simulink model "experiment_supervisor_user"  (R2026b)
settings: Solver=FixedStepDiscrete  StopTime=inf
PreLoadFcn:
  | run('experiment_supervisor_data');
model workspace (MAT data in the model file):
  Ts = 0.0001
undefined symbols (not defined in the file or in its folder): ControlModes, MCControlModes, MCMotorParamsSet
libraries: dspswit3 x1, sldrtlib x1
settings Model: DataDictionary=amcmj1.sldd  SimulationMode=accelerator  Creator=mfussi  LastModifiedBy=ksangalli
settings OptimizationCC: DefaultUnderspecifiedDataType=single  GainParamInheritBuiltInType=on  ReuseModelBlockBuffer=off  SimCompilerOptimization=on
settings DebuggingCC: ParamSuppressDoubleToSinglePrecisionLossMsg=on
settings HardwareCC: ProdHWDeviceType=Intel->x86-64 (Linux 64)  ProdLongLongMode=on
settings RTWCC: DLArmComputeVersion=19.05  Description=Simulink Desktop Real-Time  RTWCompilerOptimization=on  SystemTargetFile=sldrt.tlc  TargetLang=C++  TemplateMakefile=sldrt.tmf
settings SimulinkDesktopRealTimeCC: OptimizeReductions=on  ParMdlRefBuildCompliant=on  RealTimeExecution=kernel  TargetLangStandard=C++11 (ISO)  TargetLibSuffix=_sldrt.a  TargetPreCompLibLocation=C:\Program Files\MATLAB\R2026b\toolbox\sldrt\lib\win64

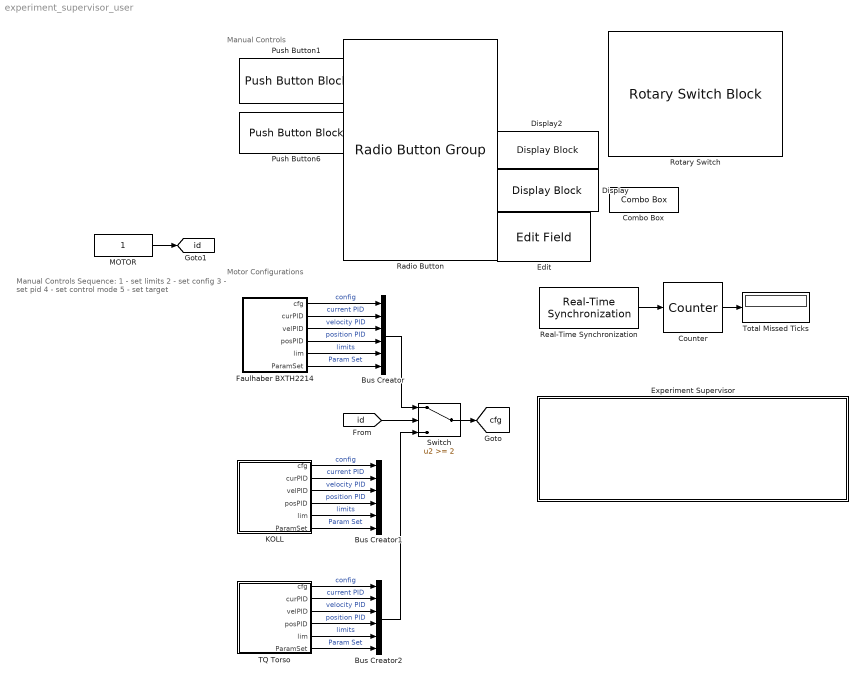
== system experiment_supervisor_user ==
  note: Manual Controls Sequence:
      | 1 - set limits
      | 2 - set config
      | 3 - set pid
      | 4 - set control mode
      | 5 - set target
  note: Motor Configurations
  note: Manual Controls
  Bus Creator : BusCreator  Inputs=6
  Bus Creator1 : BusCreator  Inputs=6
  Bus Creator2 : BusCreator  Inputs=6
  Combo Box : ComboBox  SelectedLabel=elect_vmax  UseEnumeratedDataType=on  EnumeratedDataType=MCMotorParamsSet
  Counter : dspswit3/Counter  Direction=Up  CountEvent=Rising edge  CounterSize=16 bits  MaxCount=10000  InitialCount=0  Output=Count  HitValue=32  ResetInput=off  SamplesPerFrame=1  Ts=1  CntDtype=uint16  HitDtype=Logical
  Display : DisplayBlock  Format=Integer  Transparency=1  GridColor=[1.0, 0.0, 0.0]
  Display2 : DisplayBlock  Format=Custom  Transparency=1  GridColor=[1.0, 0.0, 0.0]
  Edit : EditField  ShowInitialText=on  Alignment=Center
  Experiment Supervisor : Subsystem
  Faulhaber BXTH2214 : Subsystem
  KOLL : Subsystem
  MOTOR : Constant  OutDataTypeStr=uint32  SampleTime=0.01
  Push Button1 : PushButtonBlock  ButtonText=Send Polling CAN Msg  Icon=Triangle  IconAlignment=Right  IconOnColor=[1.0, 0.0, 1.0]  IconOffColor=[0.74901960784313726, 0.74901960784313726, 0.74901960784313726]  IconColor=On  OffValue=0.000000
  Push Button6 : PushButtonBlock  ButtonText=Send Streaming CAN Msg  ButtonType=Latch  Icon=TurnSignalRight  IconAlignment=Right  IconOnColor=[0.0, 0.0, 1.0]  IconOffColor=[0.74901960784313726, 0.74901960784313726, 0.74901960784313726]  IconColor=On  OffValue=0.000000
  Radio Button : RadioButtonGroup  LabelPosition=Hide  SelectedLabel=set-target  ButtonGroupName=Manual CAN Messages
  Real-Time Synchronization : sldrtlib/Real-Time Synchronization  SampleTime=Ts  MaxMissedTicks=inf  ShowMissedTicks=on  YieldWhenWaiting=off
  Rotary Switch : RotarySwitchBlock  LabelPosition=Hide  UseEnumeratedDataType=on  EnumeratedDataType=MCControlModes
  Switch : Switch  Threshold=2  SaturateOnIntegerOverflow=off  InputSameDT=off
  TQ Torso : Subsystem
  Total Missed Ticks : Display
      settings: Decimation=5
  tag scope: cfg=global, id=global
  wires:
  Real-Time Synchronization/1 -> Counter/1
  Faulhaber BXTH2214/1(cfg) -> Bus Creator/1  "config"
  Faulhaber BXTH2214/2(curPID) -> Bus Creator/2  "current PID"
  Faulhaber BXTH2214/3(velPID) -> Bus Creator/3  "velocity PID"
  Counter/1 -> Total Missed Ticks/1
  MOTOR/1 -> [id]
  Switch/1 -> [cfg]
  KOLL/1(cfg) -> Bus Creator1/1  "config"
  KOLL/2(curPID) -> Bus Creator1/2  "current PID"
  KOLL/3(velPID) -> Bus Creator1/3  "velocity PID"
  [id] -> Switch/2
  KOLL/5(lim) -> Bus Creator1/5  "limits"
  KOLL/4(posPID) -> Bus Creator1/4  "position PID"
  Faulhaber BXTH2214/4(posPID) -> Bus Creator/4  "position PID"
  Faulhaber BXTH2214/5(lim) -> Bus Creator/5  "limits"
  KOLL/6(ParamSet) -> Bus Creator1/6  "Param Set"
  Faulhaber BXTH2214/6(ParamSet) -> Bus Creator/6  "Param Set"
  Bus Creator/1 -> Switch/1
  TQ Torso/4(posPID) -> Bus Creator2/4  "position PID"
  TQ Torso/2(curPID) -> Bus Creator2/2  "current PID"
  TQ Torso/1(cfg) -> Bus Creator2/1  "config"
  TQ Torso/3(velPID) -> Bus Creator2/3  "velocity PID"
  TQ Torso/5(lim) -> Bus Creator2/5  "limits"
  TQ Torso/6(ParamSet) -> Bus Creator2/6  "Param Set"
  Bus Creator2/1 -> Switch/3

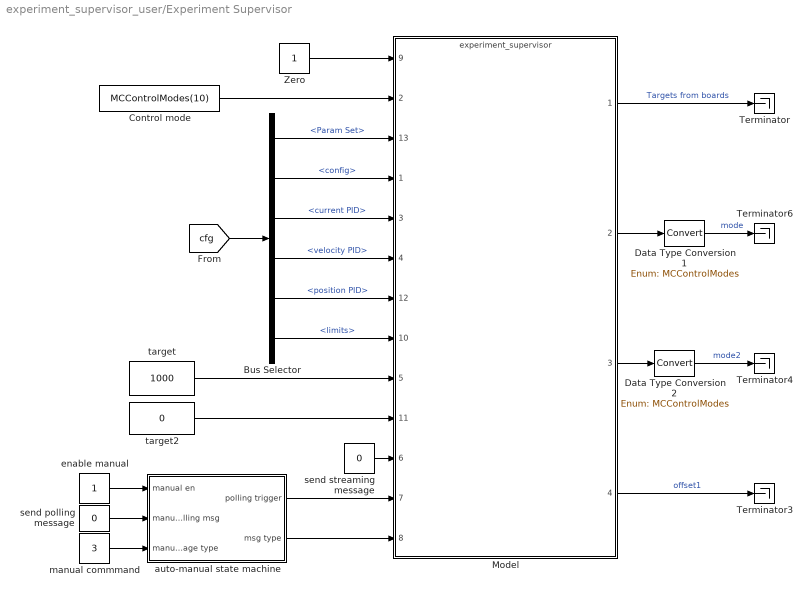
== system experiment_supervisor_user/Experiment Supervisor ==
  " Control mode" : Constant  Value=MCControlModes(10)
  Bus Selector : BusSelector  OutputSignals=Param Set,config,current PID,velocity PID,position PID,limits
  Data Type Conversion1 : DataTypeConversion  OutDataTypeStr=Enum: MCControlModes  SaturateOnIntegerOverflow=off  RndMeth=Floor
  Data Type Conversion2 : DataTypeConversion  OutDataTypeStr=Enum: MCControlModes  SaturateOnIntegerOverflow=off  RndMeth=Floor
  Model : ModelReference  ModelNameDialog=experiment_supervisor.slx  SimulationMode=Normal  ModelReferenceVersion=11.0
      settings: PortSchema="{\"entries\":[{\"content\":{\"sides\":[{\"content\":{\"connectorIds\":[\"In9\",\"In2\",\"In13\",\"In1\",\"In3\",\"In4\",\"In12\",\"In10\",\"In5\",\"In11\",\"In6\",\"In7\",\"In8\"]},\"type\":\"ConnectorPlacement.EquallySpacedRectSide\",\"uuid\":\"bfbdf898-42a5-495c-8a1e-d70d1f7414e8\"},{\"content\":{\"connectorIds\":[\"Out1\",\"Out2\",\"Out3\",\"Out4\"],\"side\":\"RIGHT\"},\"type\":\"ConnectorPlacement.EquallySpacedRectSide\",\"uuid\":\"3fb07422-e541-47fe-8bd2-34fc87b5d4e0\"},{\"content\":{\"side\":\"TOP\"},\"type\":\"ConnectorPlacement.EquallySpacedRectSide\",\"uuid\":\"cc070490-4dff-4736-882c-6ee4a91a824d\"}]},\"type\":\"ConnectorPlacement.EquallySpacedConnector\",\"uuid\":\"82f7e7bc-78f2-4fca-805f-7ff02feabc7a\"}],\"packageUris\":[\"http://schema.mathworks.com/mf0/Connector/R2020b\"],\"version\":\"1.0\"}"
  Terminator{,3..4,6} (4 alike) : Terminator
  Zero : Constant  OutDataTypeStr=Inherit: Inherit via back propagation
  auto-manual state machine : Subsystem
  enable manual : Constant  OutDataTypeStr=uint8
  manual commmand : Constant  Value=3  OutDataTypeStr=uint8
  send polling message : Constant  Value=0  OutDataTypeStr=uint8
  send streaming message : Constant  Value=0  OutDataTypeStr=Inherit: Inherit via back propagation
  target : Constant  Value=1000  OutDataTypeStr=single
  target2 : Constant  Value=0  OutDataTypeStr=single
  wires:
  Bus Selector/3 -> Model/3  "<current PID>"
  enable manual/1 -> auto-manual state machine/1(manual en)
  send polling message/1 -> auto-manual state machine/2(manual send polling msg)
  [cfg] -> Bus Selector/1
  manual commmand/1 -> auto-manual state machine/3(manual message type)
  " Control mode"/1 -> Model/2
  Bus Selector/2 -> Model/1  "<config>"
  Bus Selector/4 -> Model/4  "<velocity PID>"
  send streaming message/1 -> Model/6
  auto-manual state machine/1(polling trigger) -> Model/7
  Model/4 -> Terminator3/1  "offset1"
  auto-manual state machine/2(msg type) -> Model/8
  Model/1 -> Terminator/1  "Targets from boards"
  Model/2 -> Data Type Conversion1/1
  Data Type Conversion1/1 -> Terminator6/1  "mode"
  Zero/1 -> Model/9
  Data Type Conversion2/1 -> Terminator4/1  "mode2"
  Model/3 -> Data Type Conversion2/1
  target2/1 -> Model/11
  Bus Selector/5 -> Model/12  "<position PID>"
  target/1 -> Model/5
  Bus Selector/6 -> Model/10  "<limits>"
  Bus Selector/1 -> Model/13  "<Param Set>"

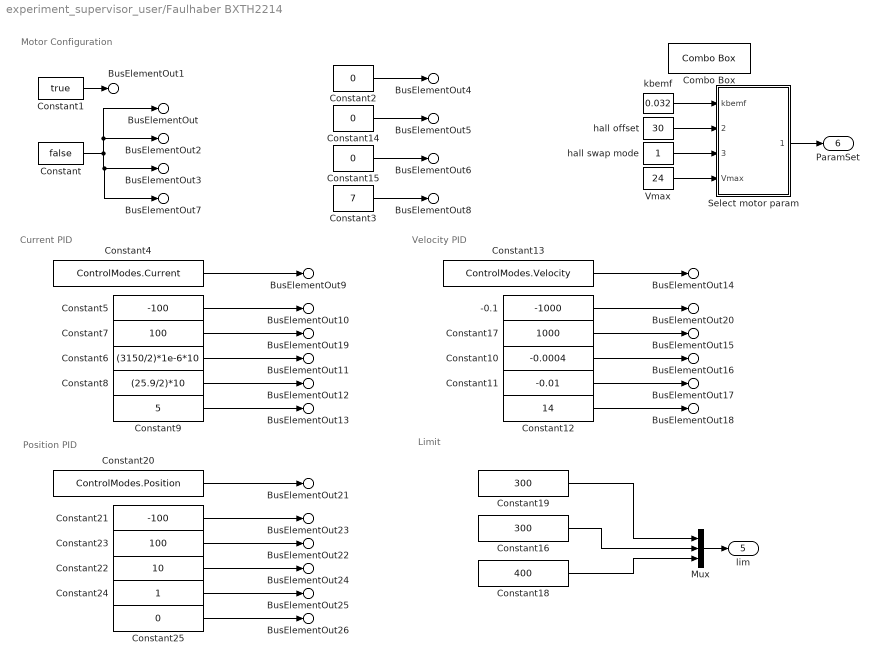
== system experiment_supervisor_user/Faulhaber BXTH2214 ==
  note: Motor Configuration
  note: Current PID
  note: Velocity PID
  note: Position PID
  note: Limit
  -0.1 : Constant  Value=-1000  OutDataTypeStr=Inherit: Inherit via back propagation
  Combo Box : ComboBox  SelectedLabel=elect_vmax  UseEnumeratedDataType=on  EnumeratedDataType=MCMotorParamsSet
  Constant : Constant  Value=false  OutDataTypeStr=Inherit: Inherit via back propagation
  Constant1 : Constant  Value=true  OutDataTypeStr=Inherit: Inherit via back propagation
  Constant10 : Constant  Value=-0.0004  OutDataTypeStr=Inherit: Inherit via back propagation
  Constant11 : Constant  Value=-0.01  OutDataTypeStr=Inherit: Inherit via back propagation
  Constant12 : Constant  Value=14  OutDataTypeStr=Inherit: Inherit via back propagation
  Constant13 : Constant  Value=ControlModes.Velocity  OutDataTypeStr=Inherit: Inherit via back propagation
  Constant{2,14..15,25} (4 alike) : Constant  Value=0  OutDataTypeStr=Inherit: Inherit via back propagation
  Constant16 : Constant  Value=300  OutDataTypeStr=Inherit: Inherit via back propagation
  Constant17 : Constant  Value=1000  OutDataTypeStr=Inherit: Inherit via back propagation
  Constant18 : Constant  Value=400  OutDataTypeStr=Inherit: Inherit via back propagation
  Constant19 : Constant  Value=300  OutDataTypeStr=Inherit: Inherit via back propagation
  Constant20 : Constant  Value=ControlModes.Position  OutDataTypeStr=Inherit: Inherit via back propagation
  Constant21 : Constant  Value=-100  OutDataTypeStr=Inherit: Inherit via back propagation
  Constant22 : Constant  Value=10  OutDataTypeStr=Inherit: Inherit via back propagation
  Constant23 : Constant  Value=100  OutDataTypeStr=Inherit: Inherit via back propagation
  Constant24 : Constant  OutDataTypeStr=Inherit: Inherit via back propagation
  Constant3 : Constant  Value=7  OutDataTypeStr=Inherit: Inherit via back propagation
  Constant4 : Constant  Value=ControlModes.Current  OutDataTypeStr=Inherit: Inherit via back propagation
  Constant5 : Constant  Value=-100  OutDataTypeStr=Inherit: Inherit via back propagation
  Constant6 : Constant  Value=(3150/2)*1e-6*10  OutDataTypeStr=Inherit: Inherit via back propagation
  Constant7 : Constant  Value=100  OutDataTypeStr=Inherit: Inherit via back propagation
  Constant8 : Constant  Value=(25.9/2)*10  OutDataTypeStr=Inherit: Inherit via back propagation
  Constant9 : Constant  Value=5  OutDataTypeStr=Inherit: Inherit via back propagation
  Mux : Mux  Inputs=3
  Select motor param : Subsystem
  Vmax : Constant  Value=24  OutDataTypeStr=single
  hall offset : Constant  Value=30  OutDataTypeStr=single
  hall swap mode : Constant  OutDataTypeStr=single
  kbemf : Constant  Value=0.032  OutDataTypeStr=single
  BusElementOut : Outport  PortName=cfg  Element=enable_verbosity
  BusElementOut1 : Outport  PortName=cfg  Element=has_hall_sens
  BusElementOut2 : Outport  PortName=cfg  Element=has_quadrature_encoder
  BusElementOut3 : Outport  PortName=cfg  Element=has_temperature_sens
  BusElementOut4 : Outport  PortName=cfg  Element=encoder_tolerance
  BusElementOut8 : Outport  PortName=cfg  Element=pole_pairs
  BusElementOut5 : Outport  PortName=cfg  Element=rotor_encoder_resolution
  BusElementOut6 : Outport  PortName=cfg  Element=rotor_index_offset
  BusElementOut7 : Outport  PortName=cfg  Element=use_index
  BusElementOut9 : Outport  Port=2  PortName=curPID  Element=type
  BusElementOut19 : Outport  Port=2  PortName=curPID  Element=OutMax
  BusElementOut10 : Outport  Port=2  PortName=curPID  Element=OutMin
  BusElementOut11 : Outport  Port=2  PortName=curPID  Element=P
  BusElementOut12 : Outport  Port=2  PortName=curPID  Element=I
  BusElementOut13 : Outport  Port=2  PortName=curPID  Element=shift_factor
  BusElementOut14 : Outport  Port=3  PortName=velPID  Element=type
  BusElementOut15 : Outport  Port=3  PortName=velPID  Element=OutMax
  BusElementOut20 : Outport  Port=3  PortName=velPID  Element=OutMin
  BusElementOut16 : Outport  Port=3  PortName=velPID  Element=P
  BusElementOut17 : Outport  Port=3  PortName=velPID  Element=I
  BusElementOut18 : Outport  Port=3  PortName=velPID  Element=shift_factor
  BusElementOut21 : Outport  Port=4  PortName=posPID  Element=type
  BusElementOut22 : Outport  Port=4  PortName=posPID  Element=OutMax
  BusElementOut23 : Outport  Port=4  PortName=posPID  Element=OutMin
  BusElementOut24 : Outport  Port=4  PortName=posPID  Element=P
  BusElementOut25 : Outport  Port=4  PortName=posPID  Element=I
  BusElementOut26 : Outport  Port=4  PortName=posPID  Element=shift_factor
  lim : Outport  Port=5
  ParamSet : Outport  Port=6
  wires:
  Constant/1 -> BusElementOut/1, BusElementOut2/1, BusElementOut7/1, BusElementOut3/1
  Constant1/1 -> BusElementOut1/1
  Constant2/1 -> BusElementOut4/1
  Constant3/1 -> BusElementOut8/1
  Constant4/1 -> BusElementOut9/1
  Constant5/1 -> BusElementOut10/1
  Constant6/1 -> BusElementOut11/1
  Constant7/1 -> BusElementOut19/1
  Constant8/1 -> BusElementOut12/1
  Constant9/1 -> BusElementOut13/1
  Constant11/1 -> BusElementOut17/1
  Constant12/1 -> BusElementOut18/1
  Constant10/1 -> BusElementOut16/1
  Constant13/1 -> BusElementOut14/1
  Constant14/1 -> BusElementOut5/1
  Constant15/1 -> BusElementOut6/1
  -0.1/1 -> BusElementOut20/1
  Constant17/1 -> BusElementOut15/1
  Constant19/1 -> Mux/1
  Constant16/1 -> Mux/2
  Mux/1 -> lim/1
  Constant18/1 -> Mux/3
  Constant24/1 -> BusElementOut25/1
  Constant25/1 -> BusElementOut26/1
  Constant21/1 -> BusElementOut23/1
  Constant23/1 -> BusElementOut22/1
  Constant20/1 -> BusElementOut21/1
  Constant22/1 -> BusElementOut24/1
  hall offset/1 -> Select motor param/2(hall offset)
  Vmax/1 -> Select motor param/4(Vmax)
  Select motor param/1(param_set) -> ParamSet/1
  hall swap mode/1 -> Select motor param/3(hall swap mode)
  kbemf/1 -> Select motor param/1(kbemf)

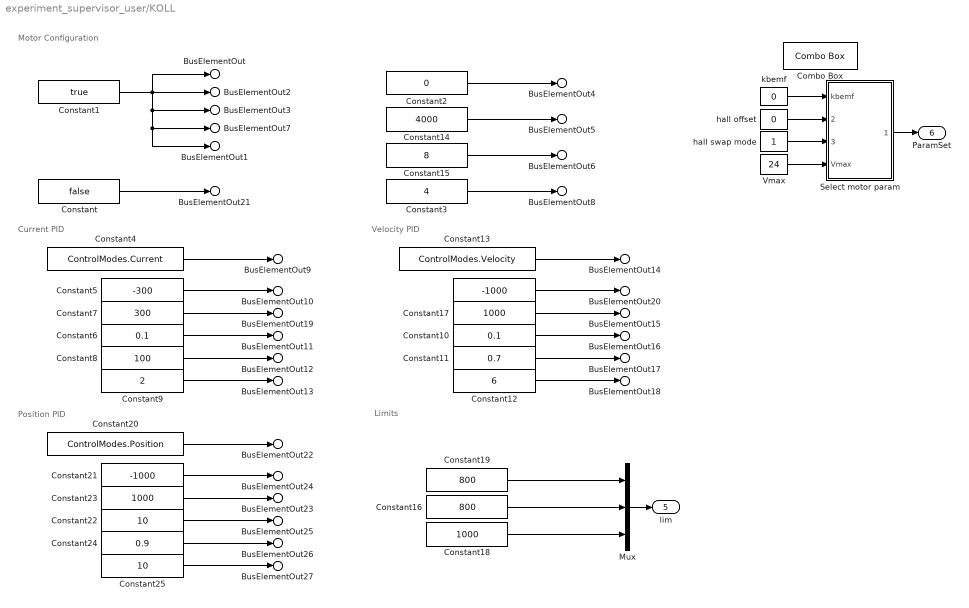
== system experiment_supervisor_user/KOLL ==
  note: Motor Configuration
  note: Current PID
  note: Velocity PID
  note: Position PID
  note: Limits
  " " : Constant  Value=-1000  OutDataTypeStr=Inherit: Inherit via back propagation
  Combo Box : ComboBox  SelectedLabel=hall  UseEnumeratedDataType=on  EnumeratedDataType=MCMotorParamsSet
  Constant : Constant  Value=false  OutDataTypeStr=Inherit: Inherit via back propagation
  Constant1 : Constant  Value=true  OutDataTypeStr=Inherit: Inherit via back propagation
  Constant10 : Constant  Value=0.1  OutDataTypeStr=Inherit: Inherit via back propagation
  Constant11 : Constant  Value=0.7  OutDataTypeStr=Inherit: Inherit via back propagation
  Constant12 : Constant  Value=6  OutDataTypeStr=Inherit: Inherit via back propagation
  Constant13 : Constant  Value=ControlModes.Velocity  OutDataTypeStr=Inherit: Inherit via back propagation
  Constant14 : Constant  Value=4000  OutDataTypeStr=Inherit: Inherit via back propagation
  Constant15 : Constant  Value=8  OutDataTypeStr=Inherit: Inherit via back propagation
  Constant16 : Constant  Value=800  OutDataTypeStr=Inherit: Inherit via back propagation
  Constant17 : Constant  Value=1000  OutDataTypeStr=Inherit: Inherit via back propagation
  Constant18 : Constant  Value=1000  OutDataTypeStr=Inherit: Inherit via back propagation
  Constant19 : Constant  Value=800  OutDataTypeStr=Inherit: Inherit via back propagation
  Constant2 : Constant  Value=0  OutDataTypeStr=Inherit: Inherit via back propagation
  Constant20 : Constant  Value=ControlModes.Position  OutDataTypeStr=Inherit: Inherit via back propagation
  Constant21 : Constant  Value=-1000  OutDataTypeStr=Inherit: Inherit via back propagation
  Constant22 : Constant  Value=10  OutDataTypeStr=Inherit: Inherit via back propagation
  Constant23 : Constant  Value=1000  OutDataTypeStr=Inherit: Inherit via back propagation
  Constant24 : Constant  Value=0.9  OutDataTypeStr=Inherit: Inherit via back propagation
  Constant25 : Constant  Value=10  OutDataTypeStr=Inherit: Inherit via back propagation
  Constant3 : Constant  Value=4  OutDataTypeStr=Inherit: Inherit via back propagation
  Constant4 : Constant  Value=ControlModes.Current  OutDataTypeStr=Inherit: Inherit via back propagation
  Constant5 : Constant  Value=-300  OutDataTypeStr=Inherit: Inherit via back propagation
  Constant6 : Constant  Value=0.1  OutDataTypeStr=Inherit: Inherit via back propagation
  Constant7 : Constant  Value=300  OutDataTypeStr=Inherit: Inherit via back propagation
  Constant8 : Constant  Value=100  OutDataTypeStr=Inherit: Inherit via back propagation
  Constant9 : Constant  Value=2  OutDataTypeStr=Inherit: Inherit via back propagation
  Mux : Mux  Inputs=3
  Select motor param : Subsystem
  Vmax : Constant  Value=24  OutDataTypeStr=single
  hall offset : Constant  Value=0  OutDataTypeStr=single
  hall swap mode : Constant  OutDataTypeStr=single
  kbemf : Constant  Value=0  OutDataTypeStr=single
  BusElementOut : Outport  PortName=cfg  Element=enable_verbosity
  BusElementOut1 : Outport  PortName=cfg  Element=has_hall_sens
  BusElementOut2 : Outport  PortName=cfg  Element=has_quadrature_encoder
  BusElementOut21 : Outport  PortName=cfg  Element=has_speed_quadrature_encoder
  BusElementOut3 : Outport  PortName=cfg  Element=has_temperature_sens
  BusElementOut4 : Outport  PortName=cfg  Element=encoder_tolerance
  BusElementOut8 : Outport  PortName=cfg  Element=pole_pairs
  BusElementOut5 : Outport  PortName=cfg  Element=rotor_encoder_resolution
  BusElementOut6 : Outport  PortName=cfg  Element=rotor_index_offset
  BusElementOut7 : Outport  PortName=cfg  Element=use_index
  BusElementOut9 : Outport  Port=2  PortName=curPID  Element=type
  BusElementOut19 : Outport  Port=2  PortName=curPID  Element=OutMax
  BusElementOut10 : Outport  Port=2  PortName=curPID  Element=OutMin
  BusElementOut11 : Outport  Port=2  PortName=curPID  Element=P
  BusElementOut12 : Outport  Port=2  PortName=curPID  Element=I
  BusElementOut13 : Outport  Port=2  PortName=curPID  Element=shift_factor
  BusElementOut14 : Outport  Port=3  PortName=velPID  Element=type
  BusElementOut15 : Outport  Port=3  PortName=velPID  Element=OutMax
  BusElementOut20 : Outport  Port=3  PortName=velPID  Element=OutMin
  BusElementOut16 : Outport  Port=3  PortName=velPID  Element=P
  BusElementOut17 : Outport  Port=3  PortName=velPID  Element=I
  BusElementOut18 : Outport  Port=3  PortName=velPID  Element=shift_factor
  BusElementOut22 : Outport  Port=4  PortName=posPID  Element=type
  BusElementOut23 : Outport  Port=4  PortName=posPID  Element=OutMax
  BusElementOut24 : Outport  Port=4  PortName=posPID  Element=OutMin
  BusElementOut25 : Outport  Port=4  PortName=posPID  Element=P
  BusElementOut26 : Outport  Port=4  PortName=posPID  Element=I
  BusElementOut27 : Outport  Port=4  PortName=posPID  Element=shift_factor
  lim : Outport  Port=5
  ParamSet : Outport  Port=6
  wires:
  Constant/1 -> BusElementOut21/1
  Constant1/1 -> BusElementOut1/1, BusElementOut7/1, BusElementOut3/1, BusElementOut2/1, BusElementOut/1
  Constant2/1 -> BusElementOut4/1
  Constant3/1 -> BusElementOut8/1
  Constant4/1 -> BusElementOut9/1
  Constant5/1 -> BusElementOut10/1
  Constant6/1 -> BusElementOut11/1
  Constant7/1 -> BusElementOut19/1
  Constant8/1 -> BusElementOut12/1
  Constant9/1 -> BusElementOut13/1
  Constant11/1 -> BusElementOut17/1
  Constant12/1 -> BusElementOut18/1
  Constant10/1 -> BusElementOut16/1
  Constant13/1 -> BusElementOut14/1
  Constant14/1 -> BusElementOut5/1
  Constant15/1 -> BusElementOut6/1
  " "/1 -> BusElementOut20/1
  Constant17/1 -> BusElementOut15/1
  Constant19/1 -> Mux/1
  Constant16/1 -> Mux/2
  Constant18/1 -> Mux/3
  Mux/1 -> lim/1
  Constant25/1 -> BusElementOut27/1
  Constant21/1 -> BusElementOut24/1
  Constant24/1 -> BusElementOut26/1
  Constant22/1 -> BusElementOut25/1
  Constant23/1 -> BusElementOut23/1
  Constant20/1 -> BusElementOut22/1
  Vmax/1 -> Select motor param/4(Vmax)
  hall swap mode/1 -> Select motor param/3(hall swap mode)
  kbemf/1 -> Select motor param/1(kbemf)
  Select motor param/1(param_set) -> ParamSet/1
  hall offset/1 -> Select motor param/2(hall offset)

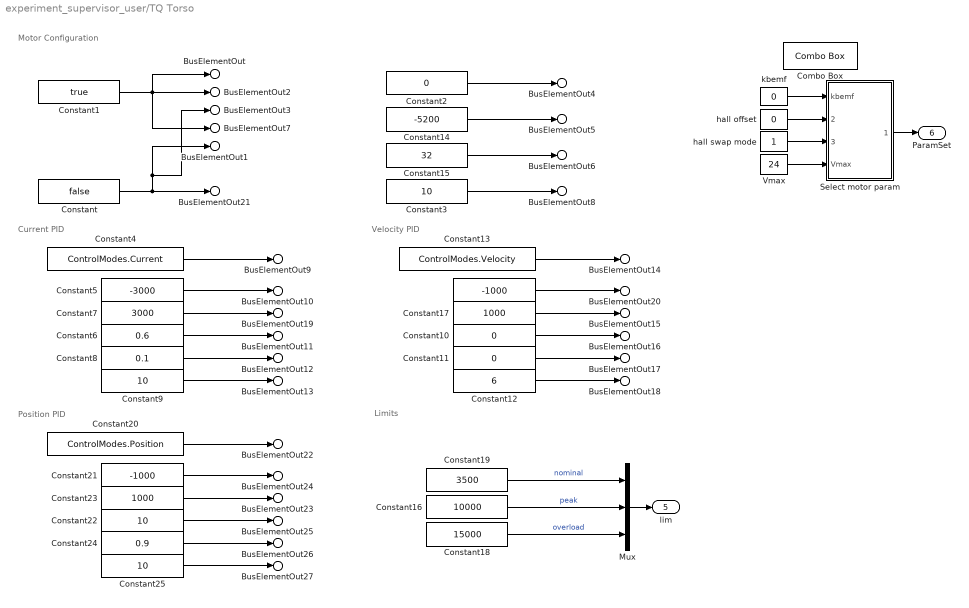
== system experiment_supervisor_user/TQ Torso ==
  note: Motor Configuration
  note: Current PID
  note: Velocity PID
  note: Position PID
  note: Limits
  " " : Constant  Value=-1000  OutDataTypeStr=Inherit: Inherit via back propagation
  Combo Box : ComboBox  SelectedLabel=elect_vmax  UseEnumeratedDataType=on  EnumeratedDataType=MCMotorParamsSet
  Constant : Constant  Value=false  OutDataTypeStr=Inherit: Inherit via back propagation
  Constant1 : Constant  Value=true  OutDataTypeStr=Inherit: Inherit via back propagation
  Constant10 : Constant  Value=0  OutDataTypeStr=Inherit: Inherit via back propagation
  Constant11 : Constant  Value=0  OutDataTypeStr=Inherit: Inherit via back propagation
  Constant12 : Constant  Value=6  OutDataTypeStr=Inherit: Inherit via back propagation
  Constant13 : Constant  Value=ControlModes.Velocity  OutDataTypeStr=Inherit: Inherit via back propagation
  Constant14 : Constant  Value=-5200  OutDataTypeStr=Inherit: Inherit via back propagation
  Constant15 : Constant  Value=32  OutDataTypeStr=Inherit: Inherit via back propagation
  Constant16 : Constant  Value=10000  OutDataTypeStr=Inherit: Inherit via back propagation
  Constant17 : Constant  Value=1000  OutDataTypeStr=Inherit: Inherit via back propagation
  Constant18 : Constant  Value=15000  OutDataTypeStr=Inherit: Inherit via back propagation
  Constant19 : Constant  Value=3500  OutDataTypeStr=Inherit: Inherit via back propagation
  Constant2 : Constant  Value=0  OutDataTypeStr=Inherit: Inherit via back propagation
  Constant20 : Constant  Value=ControlModes.Position  OutDataTypeStr=Inherit: Inherit via back propagation
  Constant21 : Constant  Value=-1000  OutDataTypeStr=Inherit: Inherit via back propagation
  Constant{3,9,22,25} (4 alike) : Constant  Value=10  OutDataTypeStr=Inherit: Inherit via back propagation
  Constant23 : Constant  Value=1000  OutDataTypeStr=Inherit: Inherit via back propagation
  Constant24 : Constant  Value=0.9  OutDataTypeStr=Inherit: Inherit via back propagation
  Constant4 : Constant  Value=ControlModes.Current  OutDataTypeStr=Inherit: Inherit via back propagation
  Constant5 : Constant  Value=-3000  OutDataTypeStr=Inherit: Inherit via back propagation
  Constant6 : Constant  Value=0.6  OutDataTypeStr=Inherit: Inherit via back propagation
  Constant7 : Constant  Value=3000  OutDataTypeStr=Inherit: Inherit via back propagation
  Constant8 : Constant  Value=0.1  OutDataTypeStr=Inherit: Inherit via back propagation
  Mux : Mux  Inputs=3
  Select motor param : Subsystem
  Vmax : Constant  Value=24  OutDataTypeStr=single
  hall offset : Constant  Value=0  OutDataTypeStr=single
  hall swap mode : Constant  OutDataTypeStr=single
  kbemf : Constant  Value=0  OutDataTypeStr=single
  BusElementOut : Outport  PortName=cfg  Element=enable_verbosity
  BusElementOut1 : Outport  PortName=cfg  Element=has_hall_sens
  BusElementOut2 : Outport  PortName=cfg  Element=has_quadrature_encoder
  BusElementOut21 : Outport  PortName=cfg  Element=has_speed_quadrature_encoder
  BusElementOut3 : Outport  PortName=cfg  Element=has_temperature_sens
  BusElementOut4 : Outport  PortName=cfg  Element=encoder_tolerance
  BusElementOut8 : Outport  PortName=cfg  Element=pole_pairs
  BusElementOut5 : Outport  PortName=cfg  Element=rotor_encoder_resolution
  BusElementOut6 : Outport  PortName=cfg  Element=rotor_index_offset
  BusElementOut7 : Outport  PortName=cfg  Element=use_index
  BusElementOut9 : Outport  Port=2  PortName=curPID  Element=type
  BusElementOut19 : Outport  Port=2  PortName=curPID  Element=OutMax
  BusElementOut10 : Outport  Port=2  PortName=curPID  Element=OutMin
  BusElementOut11 : Outport  Port=2  PortName=curPID  Element=P
  BusElementOut12 : Outport  Port=2  PortName=curPID  Element=I
  BusElementOut13 : Outport  Port=2  PortName=curPID  Element=shift_factor
  BusElementOut14 : Outport  Port=3  PortName=velPID  Element=type
  BusElementOut15 : Outport  Port=3  PortName=velPID  Element=OutMax
  BusElementOut20 : Outport  Port=3  PortName=velPID  Element=OutMin
  BusElementOut16 : Outport  Port=3  PortName=velPID  Element=P
  BusElementOut17 : Outport  Port=3  PortName=velPID  Element=I
  BusElementOut18 : Outport  Port=3  PortName=velPID  Element=shift_factor
  BusElementOut22 : Outport  Port=4  PortName=posPID  Element=type
  BusElementOut23 : Outport  Port=4  PortName=posPID  Element=OutMax
  BusElementOut24 : Outport  Port=4  PortName=posPID  Element=OutMin
  BusElementOut25 : Outport  Port=4  PortName=posPID  Element=P
  BusElementOut26 : Outport  Port=4  PortName=posPID  Element=I
  BusElementOut27 : Outport  Port=4  PortName=posPID  Element=shift_factor
  lim : Outport  Port=5
  ParamSet : Outport  Port=6
  wires:
  Constant/1 -> BusElementOut3/1, BusElementOut1/1, BusElementOut21/1
  Constant1/1 -> BusElementOut7/1, BusElementOut2/1, BusElementOut/1
  Constant2/1 -> BusElementOut4/1
  Constant3/1 -> BusElementOut8/1
  Constant4/1 -> BusElementOut9/1
  Constant5/1 -> BusElementOut10/1
  Constant6/1 -> BusElementOut11/1
  Constant7/1 -> BusElementOut19/1
  Constant8/1 -> BusElementOut12/1
  Constant9/1 -> BusElementOut13/1
  Constant11/1 -> BusElementOut17/1
  Constant12/1 -> BusElementOut18/1
  Constant10/1 -> BusElementOut16/1
  Constant13/1 -> BusElementOut14/1
  Constant14/1 -> BusElementOut5/1
  Constant15/1 -> BusElementOut6/1
  " "/1 -> BusElementOut20/1
  Constant17/1 -> BusElementOut15/1
  Constant19/1 -> Mux/1  "nominal"
  Constant16/1 -> Mux/2  "peak"
  Constant18/1 -> Mux/3  "overload"
  Mux/1 -> lim/1
  Constant25/1 -> BusElementOut27/1
  Constant21/1 -> BusElementOut24/1
  Constant24/1 -> BusElementOut26/1
  Constant22/1 -> BusElementOut25/1
  Constant23/1 -> BusElementOut23/1
  Constant20/1 -> BusElementOut22/1
  Vmax/1 -> Select motor param/4(Vmax)
  hall swap mode/1 -> Select motor param/3(hall swap mode)
  kbemf/1 -> Select motor param/1(kbemf)
  Select motor param/1(param_set) -> ParamSet/1
  hall offset/1 -> Select motor param/2(hall offset)

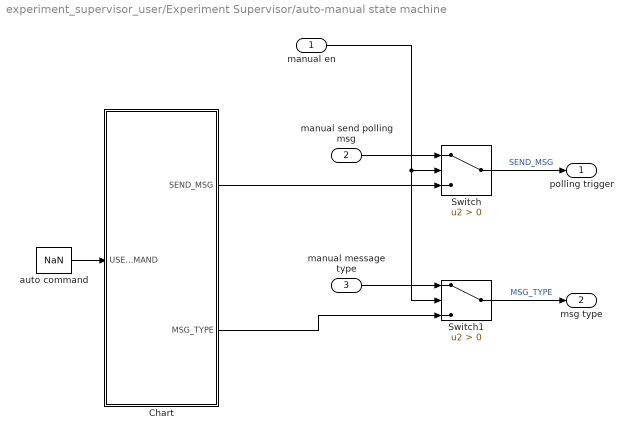
== system experiment_supervisor_user/Experiment Supervisor/auto-manual state machine ==
  manual en : Inport
  manual send polling msg : Inport  Port=2
  manual message type : Inport  Port=3
  Chart : Stateflow chart  TreatAsAtomicUnit=on
      settings: PortSchema="{\"entries\":[{\"content\":{\"sides\":[{\"content\":{\"connectorIds\":[\"In1\"]},\"type\":\"ConnectorPlacement.EquallySpacedRectSide\",\"uuid\":\"3f3ecf7a-eca8-49e2-a594-4c8df01bcae2\"},{\"content\":{\"connectorIds\":[\"Out2\",\"Out1\"],\"side\":\"RIGHT\"},\"type\":\"ConnectorPlacement.EquallySpacedRectSide\",\"uuid\":\"2e405059-6050-4daf-b42b-e1c8d6f3a572\"},{\"content\":{\"side\":\"TOP\"},\"type\":\"ConnectorPlacement.EquallySpacedRectSide\",\"uuid\":\"8705f6e5-e301-4990-b24d-44270950b42f\"}]},\"type\":\"ConnectorPlacement.EquallySpacedConnector\",\"uuid\":\"46b9b7aa-14e0-48f8-b8fe-455c7835f2bb\"}],\"packageUris\":[\"http://schema.mathworks.com/mf0/Connector/R2020b\"],\"version\":\"1.0\"}"
  Switch : Switch  Criteria=u2 > Threshold  SaturateOnIntegerOverflow=off  InputSameDT=off
  Switch1 : Switch  Criteria=u2 > Threshold  SaturateOnIntegerOverflow=off  InputSameDT=off
  auto command : Constant  Value=NaN
  polling trigger : Outport
  msg type : Outport  Port=2
  wires:
  manual en/1 -> Switch1/2, Switch/2
  manual message type/1 -> Switch1/1
  Chart/2(SEND_MSG) -> Switch/3
  Chart/1(MSG_TYPE) -> Switch1/3
  auto command/1 -> Chart/1(USER_COMMAND)
  manual send polling msg/1 -> Switch/1
  Switch1/1 -> msg type/1  "MSG_TYPE"
  Switch/1 -> polling trigger/1  "SEND_MSG"

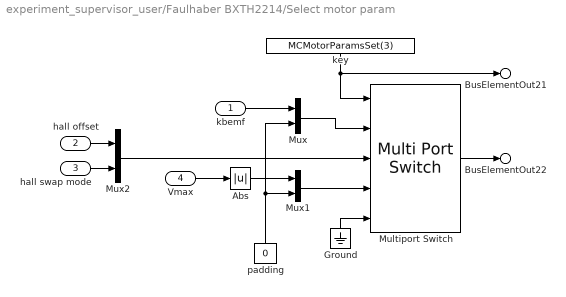
== system experiment_supervisor_user/Faulhaber BXTH2214/Select motor param ==
  kbemf : Inport
  hall offset : Inport  Port=2
  hall swap mode : Inport  Port=3
  Vmax : Inport  Port=4  OutDataTypeStr=single
  Abs : Abs  SaturateOnIntegerOverflow=off
  Ground : Ground
  Multiport Switch : MultiPortSwitch  DataPortOrder=Specify indices  DataPortIndices={MCMotorParamsSet.Kbemf, MCMotorParamsSet.hall, MCMotorParamsSet.elect_vmax}  DataPortForDefault=Additional data port  DiagnosticForDefault=None  SaturateOnIntegerOverflow=off  InputSameDT=off
  Mux : Mux  Inputs=2
  Mux1 : Mux  Inputs=2
  Mux2 : Mux  Inputs=2
  key : Constant  Value=MCMotorParamsSet(3)  OutDataTypeStr=Enum: MCMotorParamsSet
  padding : Constant  Value=0  OutDataTypeStr=single
  BusElementOut21 : Outport  PortName=param_set  Element=key
  BusElementOut22 : Outport  PortName=param_set  Element=value
  wires:
  Mux/1 -> Multiport Switch/2
  kbemf/1 -> Mux/1
  Mux2/1 -> Multiport Switch/3
  Mux1/1 -> Multiport Switch/4
  Ground/1 -> Multiport Switch/5
  padding/1 -> Mux/2, Mux1/2
  hall offset/1 -> Mux2/1
  hall swap mode/1 -> Mux2/2
  Vmax/1 -> Abs/1
  key/1 -> BusElementOut21/1, Multiport Switch/1
  Multiport Switch/1 -> BusElementOut22/1
  Abs/1 -> Mux1/1

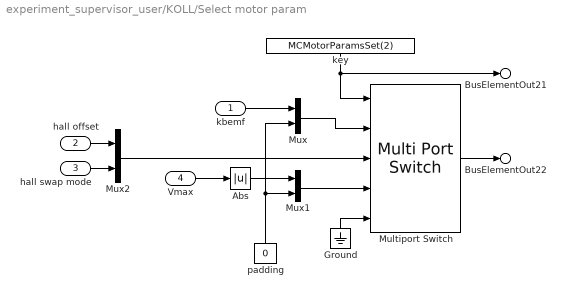
== system experiment_supervisor_user/KOLL/Select motor param ==
  kbemf : Inport
  hall offset : Inport  Port=2
  hall swap mode : Inport  Port=3
  Vmax : Inport  Port=4  OutDataTypeStr=single
  Abs : Abs  SaturateOnIntegerOverflow=off
  Ground : Ground
  Multiport Switch : MultiPortSwitch  DataPortOrder=Specify indices  DataPortIndices={MCMotorParamsSet.Kbemf, MCMotorParamsSet.hall, MCMotorParamsSet.elect_vmax}  DataPortForDefault=Additional data port  DiagnosticForDefault=None  SaturateOnIntegerOverflow=off  InputSameDT=off
  Mux : Mux  Inputs=2
  Mux1 : Mux  Inputs=2
  Mux2 : Mux  Inputs=2
  key : Constant  Value=MCMotorParamsSet(2)  OutDataTypeStr=Enum: MCMotorParamsSet
  padding : Constant  Value=0  OutDataTypeStr=single
  BusElementOut21 : Outport  PortName=param_set  Element=key
  BusElementOut22 : Outport  PortName=param_set  Element=value
  wires:
  Mux/1 -> Multiport Switch/2
  kbemf/1 -> Mux/1
  Mux2/1 -> Multiport Switch/3
  Mux1/1 -> Multiport Switch/4
  Ground/1 -> Multiport Switch/5
  padding/1 -> Mux/2, Mux1/2
  hall offset/1 -> Mux2/1
  hall swap mode/1 -> Mux2/2
  Vmax/1 -> Abs/1
  key/1 -> BusElementOut21/1, Multiport Switch/1
  Multiport Switch/1 -> BusElementOut22/1
  Abs/1 -> Mux1/1

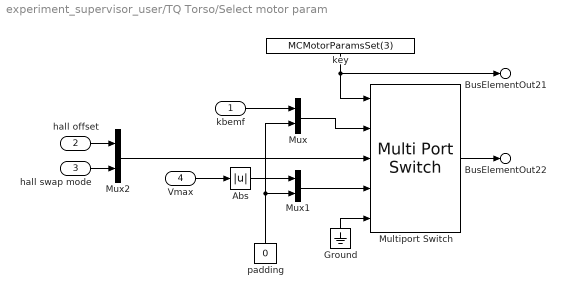
== system experiment_supervisor_user/TQ Torso/Select motor param ==
  kbemf : Inport
  hall offset : Inport  Port=2
  hall swap mode : Inport  Port=3
  Vmax : Inport  Port=4  OutDataTypeStr=single
  Abs : Abs  SaturateOnIntegerOverflow=off
  Ground : Ground
  Multiport Switch : MultiPortSwitch  DataPortOrder=Specify indices  DataPortIndices={MCMotorParamsSet.Kbemf, MCMotorParamsSet.hall, MCMotorParamsSet.elect_vmax}  DataPortForDefault=Additional data port  DiagnosticForDefault=None  SaturateOnIntegerOverflow=off  InputSameDT=off
  Mux : Mux  Inputs=2
  Mux1 : Mux  Inputs=2
  Mux2 : Mux  Inputs=2
  key : Constant  Value=MCMotorParamsSet(3)  OutDataTypeStr=Enum: MCMotorParamsSet
  padding : Constant  Value=0  OutDataTypeStr=single
  BusElementOut21 : Outport  PortName=param_set  Element=key
  BusElementOut22 : Outport  PortName=param_set  Element=value
  wires:
  Mux/1 -> Multiport Switch/2
  kbemf/1 -> Mux/1
  Mux2/1 -> Multiport Switch/3
  Mux1/1 -> Multiport Switch/4
  Ground/1 -> Multiport Switch/5
  padding/1 -> Mux/2, Mux1/2
  hall offset/1 -> Mux2/1
  hall swap mode/1 -> Mux2/2
  Vmax/1 -> Abs/1
  key/1 -> BusElementOut21/1, Multiport Switch/1
  Multiport Switch/1 -> BusElementOut22/1
  Abs/1 -> Mux1/1

== stateflow chart experiment_supervisor_user/Experiment Supervisor/auto-manual state machine/Chart ==
  state RESET_IDLE
    entry:
    SEND_MSG=1;
    on after(1, sec):
    SEND_MSG=0;
  state WAIT_LIMITS
    entry:
    SEND_MSG=1;
    on after(1, sec):
    SEND_MSG=0;
  state IDLE
    entry:
    SEND_MSG=1;
    on after(1 , sec):
    SEND_MSG=0;
  state STARTED
    entry:
    SEND_MSG=1;
    on after(1 , sec):
    SEND_MSG=0;
  state WAIT_CTRL_MODE
    entry:
    SEND_MSG=1;
    on after(1,sec):
    SEND_MSG=0;
  (default) -> RESET_IDLE
  STARTED -> RESET_IDLE [order 3] : [USER_COMMAND == 2]
      | {MSG_TYPE = 1;}
  RESET_IDLE -> WAIT_LIMITS [order 1] : [USER_COMMAND == 1]
      | {MSG_TYPE = 4;}
  IDLE -> RESET_IDLE [order 2] : [USER_COMMAND == 2]
      | {MSG_TYPE=1;}
  WAIT_LIMITS -> RESET_IDLE [order 2] : [USER_COMMAND == 2]
      | {MSG_TYPE = 1;}
  RESET_IDLE -> RESET_IDLE [order 2] : [USER_COMMAND == 2]
      | {MSG_TYPE=1;}
  WAIT_CTRL_MODE -> RESET_IDLE [order 2] : [USER_COMMAND == 2]
      | {MSG_TYPE = 1;}
  IDLE -> IDLE [order 3] : [USER_COMMAND == 0 ]
      | {MSG_TYPE=1;}
  WAIT_LIMITS -> WAIT_CTRL_MODE [order 1] : after(2, sec){MSG_TYPE = 2;}
  STARTED -> IDLE [order 1] : [USER_COMMAND == 0 ]
      | {MSG_TYPE=1;}
  IDLE -> WAIT_CTRL_MODE [order 1] : [USER_COMMAND == 1]
      | {MSG_TYPE = 2;}
  WAIT_CTRL_MODE -> STARTED [order 1] : after(2, sec){MSG_TYPE=3;}
  STARTED -> STARTED [order 2] : [USER_COMMAND == 1]{MSG_TYPE = 3;}
  data: MSG_TYPE output uint8 =uint8(1); USER_COMMAND input; SEND_MSG output uint8 =uint8(0)
